simulink model "duck_sim"  (R2026b)
settings: Solver=FixedStepDiscrete  StopTime=5  FixedStep=DT_PLANT
PreLoadFcn:
  | startup_duck; load(fullfile(DUCK_PROJ,'matlab','duck_params.mat'));
values from neighbouring files (symbols this model uses):
  ALPHA = 0.5/(0.5+DT_CTRL)    (= 0.980392156863)    [duck_numbers.m]    (also in duck_params.mat)
  ANKLE_MAP = zeros(14,1);  ANKLE_MAP(IDX_L_ANKLE) = 1;  ANKLE_MAP(IDX_R_ANKLE) = -1    [build_duck_sim.m]    (also in duck_numbers.m; duck_params.mat = [0 0 0 0 1 0 0 0 0 0 0 0 ... (14 elements, 14x1)])
  balance_on = 1    [duck_numbers.m]    (also in duck_params.mat)
  C = [mdl '/Controller']    [build_duck_sim.m]
  DT_CTRL = 0.01    [duck_numbers.m]    (also in duck_params.mat)
  DT_PLANT = S.timestep    [duck_numbers.m]    (also in duck_params.mat = 0.002)
  HOME = S.home(:)    [duck_numbers.m]    (also in duck_params.mat = [0 -0.0872664625997 -0.457924 -0.00494 0.452984 0.3490658503)
  K_D = Kd/kp_total    [duck_numbers.m]    (also in duck_params.mat = 0.185741871987)
  K_TH = Kp/kp_total    [duck_numbers.m]    (also in duck_params.mat = 2.33868990942)
  push_F = 0    [duck_numbers.m]    (also in duck_params.mat)
  SAT_ANKLE = 0.25    [duck_numbers.m]    (also in duck_params.mat)
libraries: mjLib x1
settings Model: Creator=caide  LastModifiedBy=caide

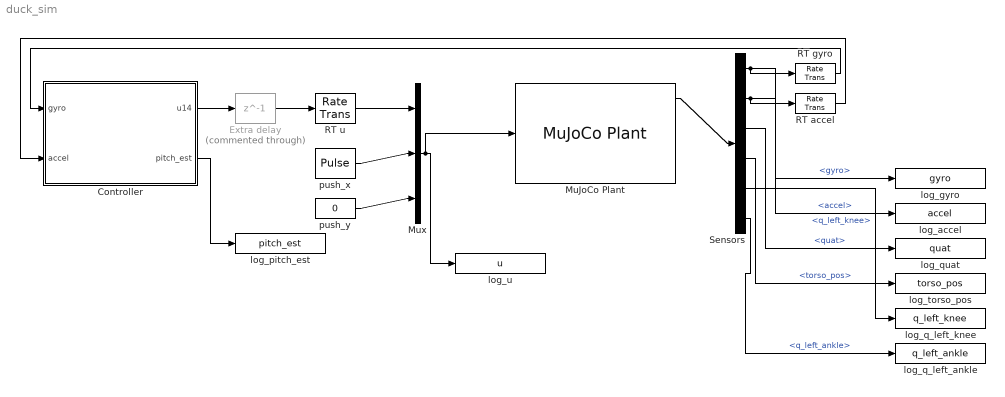
== system duck_sim ==
  Controller : Subsystem  TreatAsAtomicUnit=on  SystemSampleTime=DT_CTRL
  Extra delay : Delay  Commented=through  DelayLength=1  InitialCondition=HOME  SampleTime=DT_CTRL
  MuJoCo Plant : mjLib/MuJoCo Plant  controlBus=[]  sensorBus=mj_bus_sensor_7979902499018342666  controlLength=[]  sensorLength=[]  rgbLength=[]  depthLength=[]  sampleTime=0.002  xmlFileRel=C:\dev\duckling_sim\model\duck_v3_scene.xml  xmlFile=C:\dev\duckling_sim\model\duck_v3_scene.xml  renderingType=Global  vsync=off  visualFPS=60  zoomLevel=1  znear=0.02  zfar=100  cameraSampleTime=0.020  rgbOutOption=on  depthOutOption=on  controlInterfaceType=Vector
      settings: SourceProductName=MuJoCo Simulator
  Mux : Mux  Inputs=3
  RT accel : RateTransition  OutPortSampleTime=DT_CTRL
  RT gyro : RateTransition  OutPortSampleTime=DT_CTRL
  RT u : RateTransition  InitialCondition=HOME  OutPortSampleTime=DT_PLANT
  Sensors : BusSelector  OutputSignals=gyro,accel,quat,torso_pos,q_left_knee,q_left_ankle
  log_accel : ToWorkspace  VariableName=accel  SaveFormat=Timeseries  SampleTime=-1
  log_gyro : ToWorkspace  VariableName=gyro  SaveFormat=Timeseries  SampleTime=-1
  log_pitch_est : ToWorkspace  VariableName=pitch_est  SaveFormat=Timeseries  SampleTime=-1
  log_q_left_ankle : ToWorkspace  VariableName=q_left_ankle  SaveFormat=Timeseries  SampleTime=-1
  log_q_left_knee : ToWorkspace  VariableName=q_left_knee  SaveFormat=Timeseries  SampleTime=-1
  log_quat : ToWorkspace  VariableName=quat  SaveFormat=Timeseries  SampleTime=-1
  log_torso_pos : ToWorkspace  VariableName=torso_pos  SaveFormat=Timeseries  SampleTime=-1
  log_u : ToWorkspace  VariableName=u  SaveFormat=Timeseries  SampleTime=-1
  push_x : DiscretePulseGenerator  Amplitude=push_F  Period=round(100/DT_PLANT)  PulseWidth=round(0.05/DT_PLANT)  PhaseDelay=round(1/DT_PLANT)  SampleTime=DT_PLANT
  push_y : Constant  Value=0  SampleTime=DT_PLANT
  wires:
  MuJoCo Plant/1 -> Sensors/1
  Sensors/1 -> RT gyro/1, log_gyro/1  "<gyro>"
  Sensors/2 -> RT accel/1, log_accel/1  "<accel>"
  RT gyro/1 -> Controller/1(gyro)
  RT accel/1 -> Controller/2(accel)
  Controller/1(u14) -> Extra delay/1
  Extra delay/1 -> RT u/1
  RT u/1 -> Mux/1
  push_x/1 -> Mux/2
  push_y/1 -> Mux/3
  Mux/1 -> MuJoCo Plant/1, log_u/1
  Sensors/3 -> log_quat/1  "<quat>"
  Sensors/4 -> log_torso_pos/1  "<torso_pos>"
  Sensors/5 -> log_q_left_knee/1  "<q_left_knee>"
  Sensors/6 -> log_q_left_ankle/1  "<q_left_ankle>"
  Controller/2(pitch_est) -> log_pitch_est/1

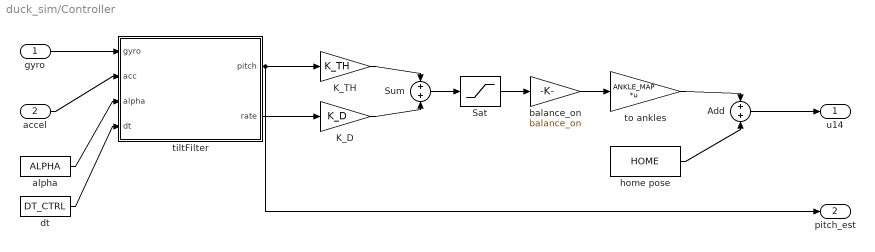
== system duck_sim/Controller ==
  gyro : Inport
  accel : Inport  Port=2
  Add : Sum
  K_D : Gain  Gain=K_D
  K_TH : Gain  Gain=K_TH
  Sat : Saturate  UpperLimit=SAT_ANKLE  LowerLimit=-SAT_ANKLE
  Sum : Sum
  alpha : Constant  Value=ALPHA
  balance_on : Gain  Gain=balance_on
  dt : Constant  Value=DT_CTRL
  home pose : Constant  Value=HOME
  tiltFilter : MATLAB Function  TreatAsAtomicUnit=on
  to ankles : Gain  Gain=ANKLE_MAP  Multiplication=Matrix(K*u)
  u14 : Outport
  pitch_est : Outport  Port=2
  wires:
  gyro/1 -> tiltFilter/1(gyro)
  accel/1 -> tiltFilter/2(acc)
  alpha/1 -> tiltFilter/3(alpha)
  dt/1 -> tiltFilter/4(dt)
  tiltFilter/1(pitch) -> K_TH/1, pitch_est/1
  tiltFilter/2(rate) -> K_D/1
  K_TH/1 -> Sum/1
  K_D/1 -> Sum/2
  Sum/1 -> Sat/1
  Sat/1 -> balance_on/1
  balance_on/1 -> to ankles/1
  to ankles/1 -> Add/1
  home pose/1 -> Add/2
  Add/1 -> u14/1

== matlab function duck_sim/Controller/tiltFilter ==
  data: gyro input; pitch output; acc input; alpha input; dt input; rate output
function [pitch, rate] = tiltFilter(gyro, acc, alpha, dt)
%#codegen
% Complementary filter: gyro is accurate short-term, accelerometer does not drift.
persistent th
if isempty(th), th = 0; end
accPitch = atan2(-acc(1), acc(3));        % + = leaning forward (nose down)
th    = alpha*(th + gyro(2)*dt) + (1 - alpha)*accPitch;
pitch = th;         % rad
rate  = gyro(2);    % rad/s
end
